simulink model "Powertrain"  (R2022a)
settings: Solver=FixedStepAuto  StartTime=0.0  StopTime=inf  FixedStep=1  RelTol=1e-3
model workspace (MAT data in the model file):
  Velocity_kmph = Simulink.Parameter
  Velocity_kmph.DataType = 'auto'
  Velocity_kmph.Complexity = 'real'
  Velocity_kmph.Dimensions = [0 0]
values from neighbouring files (symbols this model uses):
  Batt_Capacity = 66.2    [Imports.m]
  Batt_Energy = 24000    [Imports.m]
  Cd = 0.28    [Imports.m]
  Cell_SOC = Cell(:,3)    [Imports.m]
  Cell_Volt = Cell(:,2)    [Imports.m]
  Crf = 0.015    [Imports.m]
  Fa = 3.8056    [Imports.m]
  GR = 7.9377    [Imports.m]
  GVM = Mv+Md    (= 1710.665)    [Imports.m]
  GVW = GVM*g    (= 16781.62365)    [Imports.m]
  HSOC = 80    [Imports.m]
  Ir = 0.0023    [Imports.m]
  K_EMF = 0.238    [Imports.m]
  K_T = 0.195    [Imports.m]
  LSOC = 20    [Imports.m]
  M_C_Regen_Eff = M_C_Regen(:,2:16)    [Imports.m]
  M_C_Regen_Speed = M_C_Regen(:,1)    [Imports.m]
  M_C_Regen_Torque = M_C_Regen(:,17)    [Imports.m]
  M_Controller_Eff = M_Controller(:,2:16)    [Imports.m]
  M_Controller_Speed = M_Controller(:,1)    [Imports.m]
  M_Controller_Torque = M_Controller(:,17)    [Imports.m]
  Max_Battery_Regen_Current = Max_Regen_Current*Np    (= 66.2)    [Imports.m]
  Motor_Eff = Motor(:,2:16)    [Imports.m]
  Motor_Regen_Eff = Motor_Regen(:,2:16)    [Imports.m]
  Motor_Regen_Speed = Motor_Regen(:,1)    [Imports.m]
  Motor_Regen_Torque = Motor_Regen(:,17)    [Imports.m]
  Motor_Speed = Motor(:,1)    [Imports.m]
  Motor_Torque = Motor(:,17)    [Imports.m]
  Ns = 96    [Imports.m]
  R_Arm = 0.00567    [Imports.m]
  rho = 1.225    [Imports.m]
  Rw = 0.2032    [Imports.m]
  Teff = 0.89    [Imports.m]
settings Model: Creator=goodbox  LastModifiedBy=sujee
settings SolverCC: AlgebraicLoopSolver=TrustRegion
settings DebuggingCC: UnconnectedInputMsg=warning  UnconnectedOutputMsg=warning  UnconnectedLineMsg=warning  SFMachineParentedDataDiag=warning

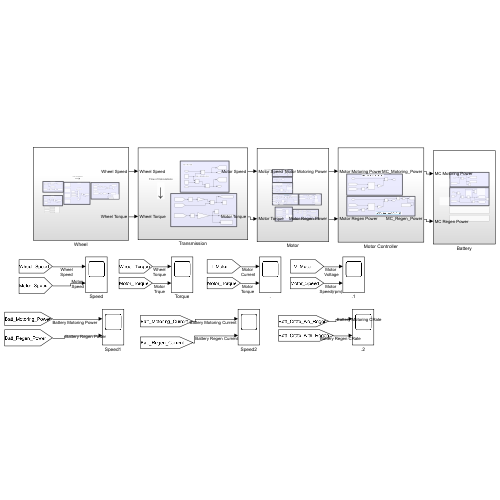
[thumbnail: Simulink's stored preview of the top-level diagram]
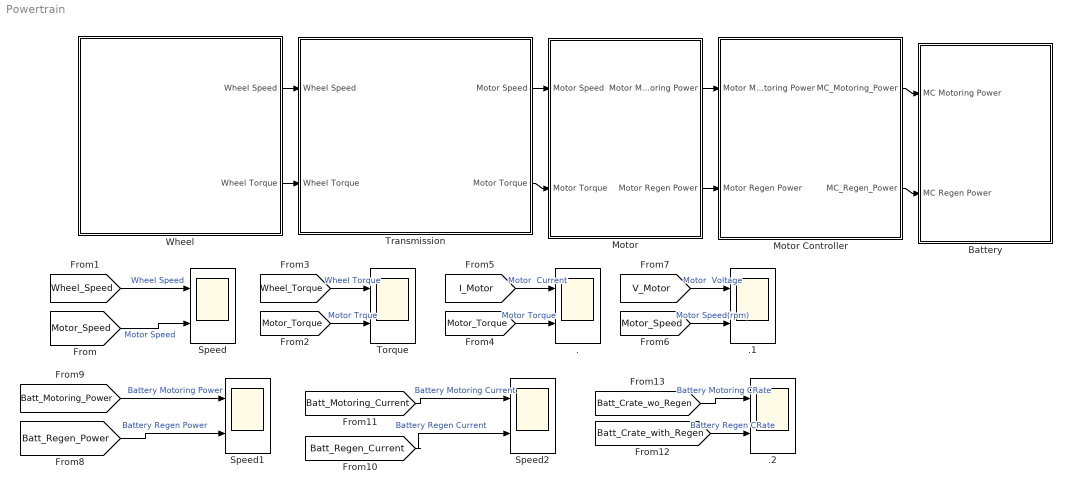
== system Powertrain ==
  . : Scope  NumInputPorts=2
  .1 : Scope  NumInputPorts=2
  .2 : Scope  NumInputPorts=2
  Battery : Subsystem
  Motor : Subsystem
  Motor Controller : Subsystem
  Speed : Scope  NumInputPorts=2
  Speed1 : Scope  NumInputPorts=2
  Speed2 : Scope  NumInputPorts=2
  Torque : Scope  NumInputPorts=2
  Transmission : Subsystem
  Wheel : Subsystem
  wires:
  Wheel/1(Wheel Speed) -> Transmission/1(Wheel Speed)
  Wheel/2(Wheel Torque) -> Transmission/2(Wheel Torque)
  [Wheel_Speed] -> Speed/1  "Wheel Speed"
  [Motor_Speed] -> Speed/2  "Motor Speed"
  [Motor_Torque] -> Torque/2  "Motor Trque"
  [Wheel_Torque] -> Torque/1  "Wheel Torque"
  Transmission/1(Motor Speed) -> Motor/1(Motor Speed)
  Transmission/2(Motor Torque) -> Motor/2(Motor Torque)
  [I_Motor] -> ./1  "Motor  Current"
  [Motor_Torque] -> ./2  "Motor Torque"
  [Motor_Speed] -> .1/2  "Motor Speed(rpm)"
  [V_Motor] -> .1/1  "Motor  Voltage"
  Motor/1(Motor Motoring Power) -> Motor Controller/1(Motor Motoring Power)
  Motor/2(Motor Regen Power) -> Motor Controller/2(Motor Regen Power)
  Motor Controller/2(MC_Regen_Power) -> Battery/2(MC Regen Power)
  Motor Controller/1(MC_Motoring_Power) -> Battery/1(MC Motoring Power)
  [Batt_Regen_Power] -> Speed1/2  "Battery Regen Power"
  [Batt_Motoring_Power] -> Speed1/1  "Battery Motoring Power"
  [Batt_Motoring_Current] -> Speed2/1  "Battery Motoring Current"
  [Batt_Regen_Current] -> Speed2/2  "Battery Regen Current"
  [Batt_Crate_wo_Regen] -> .2/1  "Battery Motoring CRate"
  [Batt_Crate_with_Regen] -> .2/2  "Battery Regen CRate"

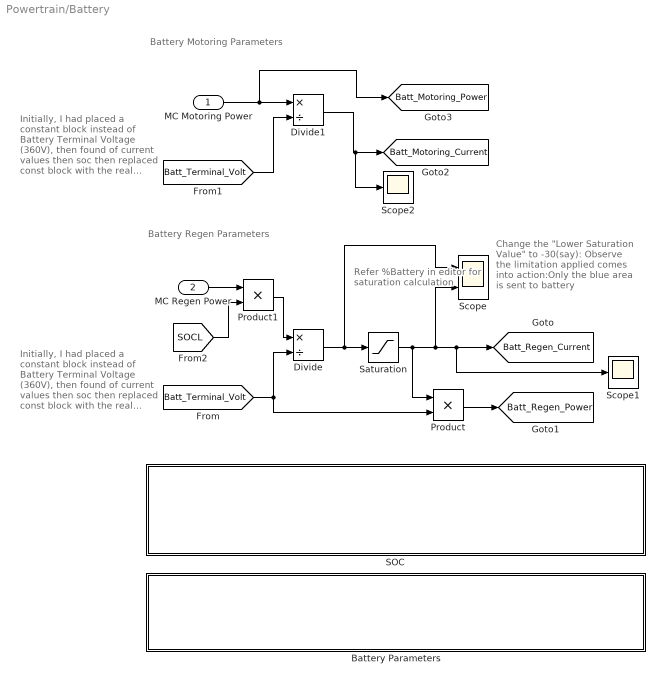
== system Powertrain/Battery ==
  note: Initially, I had placed a constant block instead of Battery Terminal Voltage (360V), then found of current values then soc then replaced const block with the real battery terminal voltage...
  note: Battery Motoring Parameters
  note: Battery Regen Parameters
  note: Refer %Battery in editor for saturation calculation
  note: Change the "Lower Saturation Value" to -30(say): Observe the limitation applied comes into action:Only the blue area is sent to battery
  note: Initially, I had placed a constant block instead of Battery Terminal Voltage (360V), then found of current values then soc then replaced const block with the real battery terminal voltage...
  MC Motoring Power : Inport
  MC Regen Power : Inport  Port=2
  Battery Parameters : Subsystem
  Divide : Product  Inputs=*/
  Divide1 : Product  Inputs=*/
  Product : Product
  Product1 : Product
  SOC : Subsystem
  Saturation : Saturate  UpperLimit=0  LowerLimit=-(Max_Battery_Regen_Current)
  Scope : Scope  NumInputPorts=2
  Scope1 : Scope
  Scope2 : Scope
  tag scope: Batt_Motoring_Current=global, Batt_Motoring_Power=global, Batt_Regen_Current=global, Batt_Regen_Power=global
  wires:
  [Batt_Terminal_Volt] -> Product/2, Divide/2
  Divide/1 -> Scope/1, Saturation/1
  Saturation/1 -> Scope/2, Scope1/1, [Batt_Regen_Current], Product/1
  Product/1 -> [Batt_Regen_Power]
  MC Motoring Power/1 -> [Batt_Motoring_Power], Divide1/1
  [Batt_Terminal_Volt] -> Divide1/2
  Divide1/1 -> Scope2/1, [Batt_Motoring_Current]
  Product1/1 -> Divide/1
  MC Regen Power/1 -> Product1/1
  [SOCL] -> Product1/2

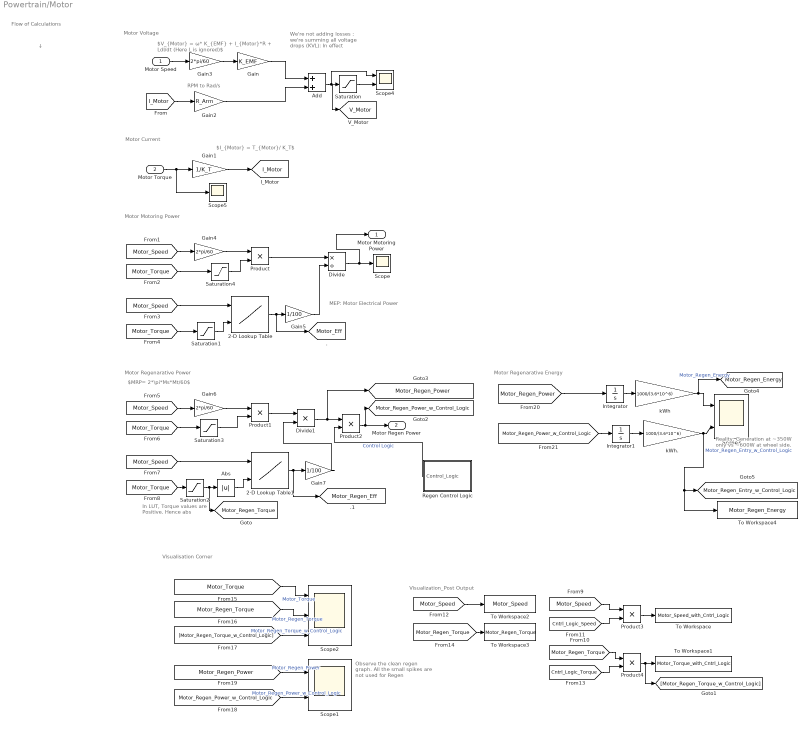
== system Powertrain/Motor ==
  note: Visualization_Post Output
  note: Motor Regenarative Energy
  note: Visualisation Corner
  note: Observe the clean regen graph. All the small spikes are not used for Regen
  note: MEP: Motor Electrical Power
  note: In LUT, Torque values are Positive. Hence abs
  note: $MRP= 2*\pi*Ms*Mt/60$
  note: Motor Motoring Power
  note: Motor Current
  note: Motor Voltage
  note: We're not adding losses : we're summing all voltage drops (KVL): In effect
  note: RPM to Rad/s
  note: $I_{Motor} = T_{Motor}/ K_T$
  note: $V_{Motor} = ω* K_{EMF} + I_{Motor}*R + LdI/dt (Here L is ignored)$
  note: Motor Regenarative Power
  note: ↓
  note: Flow of Calculations
  note: Reality: Generation at ~350W only vs ~600W at wheel side.
  Motor Speed : Inport
  Motor Torque : Inport  Port=2
  2-D Lookup Table : Lookup_n-D  BreakpointsForDimension1=Motor_Speed  BreakpointsForDimension2=Motor_Torque  Table=Motor_Eff  InternalRulePriority=Speed  RndMeth=Simplest
      settings: InputPortMap=u0,u1
  2-D Lookup Table1 : Lookup_n-D  BreakpointsForDimension1=Motor_Regen_Speed  BreakpointsForDimension2=Motor_Regen_Torque  Table=Motor_Regen_Eff  InternalRulePriority=Speed  RndMeth=Simplest
      settings: InputPortMap=u0,u1
  Abs : Abs  SaturateOnIntegerOverflow=off
  Add : Sum
  Divide : Product  Inputs=*/
  Divide1 : Product  Inputs=**
  Gain : Gain  Gain=K_EMF
  Gain1 : Gain  Gain=1/K_T
  Gain2 : Gain  Gain=R_Arm
  Gain3 : Gain  Gain=2*pi/60
  Gain4 : Gain  Gain=2*pi/60
  Gain5 : Gain  Gain=1/100
  Gain6 : Gain  Gain=2*pi/60
  Gain7 : Gain  Gain=1/100
  Integrator : Integrator
  Integrator1 : Integrator
  Product{,1..4} (5 alike) : Product
  Regen Control Logic : Subsystem
      settings: PortSchema="{\"entries\":[{\"content\":{\"sides\":[{\"content\":{\"connectorIds\":[\"Out1\"]},\"type\":\"ConnectorPlacement.EquallySpacedRectSide\",\"uuid\":\"9e0a81c3-7851-4a2a-9294-227ed6cb1b10\"},{\"content\":{\"connectorIds\":[],\"side\":\"RIGHT\"},\"type\":\"ConnectorPlacement.EquallySpacedRectSide\",\"uuid\":\"e9ef44a6-e013-44a9-929d-6b26e6cf2f5f\"},{\"content\":{\"connectorIds\":[],\"side\":\"TOP\"},\"type\":\"ConnectorPlacement.EquallySpacedRectSide\",\"uuid\":\"caa0c9f2-8ad3-43be-baf4-e18c04196c42\"}]},\"type\":\"ConnectorPlacement.EquallySpacedConnector\",\"uuid\":\"14208f40-628f-4a93-bd22-09b3f37d5a54\"}],\"packageUris\":[\"http://schema.mathworks.com/mf0/Connector/R2020b\"],\"version\":\"1.0\"}"
  Saturation : Saturate  UpperLimit=inf  LowerLimit=0
  Saturation1 : Saturate  UpperLimit=inf  LowerLimit=0
  Saturation2 : Saturate  UpperLimit=0  LowerLimit=-inf
  Saturation3 : Saturate  UpperLimit=0  LowerLimit=-inf
  Saturation4 : Saturate  UpperLimit=inf  LowerLimit=0
  Scope : Scope
  Scope1 : Scope  NumInputPorts=2
  Scope2 : Scope  NumInputPorts=3
  Scope3 : Scope  NumInputPorts=2
  Scope4 : Scope  NumInputPorts=2
  Scope5 : Scope
  To Workspace : ToWorkspace  VariableName=Motor_Speed_with_Cntrl_Logic  SaveFormat=Timeseries  SampleTime=-1
  To Workspace1 : ToWorkspace  VariableName=Motor_Torque_with_Cntrl_Logic  SaveFormat=Timeseries  SampleTime=-1
  To Workspace2 : ToWorkspace  VariableName=Motor_Speed  SaveFormat=Timeseries  SampleTime=-1
  To Workspace3 : ToWorkspace  VariableName=Motor_Regen_Torque  SaveFormat=Timeseries  SampleTime=-1
  To Workspace4 : ToWorkspace  VariableName=Motor_Regen_Energy  SaveFormat=Timeseries  SampleTime=-1
  kWh : Gain  Gain=1000/(3.6*10^6)
  kWh. : Gain  Gain=1000/(3.6*10^6)
  Motor Motoring Power : Outport
  Motor Regen Power : Outport  Port=2
  tag scope: I_Motor=global, Motor_Eff=global, Motor_Regen_Eff=global, Motor_Regen_Energy=global, Motor_Regen_Entry_w_Control_Logic=global, Motor_Regen_Power=global, Motor_Regen_Power_w_Control_Logic=global, Motor_Regen_Torque=global, V_Motor=global
  wires:
  Gain/1 -> Add/1
  Motor Torque/1 -> Scope5/1, Gain1/1
  Gain1/1 -> [I_Motor]
  [I_Motor] -> Gain2/1
  Gain2/1 -> Add/2
  Motor Speed/1 -> Gain3/1
  Gain3/1 -> Gain/1
  Add/1 -> Scope4/1, Saturation/1, [V_Motor]
  [Motor_Speed] -> Gain4/1
  Gain4/1 -> Product/1
  [Motor_Speed] -> 2-D Lookup Table/1
  2-D Lookup Table/1 -> [Motor_Eff], Gain5/1
  Product/1 -> Divide/1
  Gain5/1 -> Divide/2
  [Motor_Torque] -> Saturation1/1
  Saturation1/1 -> 2-D Lookup Table/2
  Divide/1 -> Scope/1, Motor Motoring Power/1
  [Motor_Speed] -> 2-D Lookup Table1/1
  Product1/1 -> Divide1/1
  2-D Lookup Table1/1 -> [Motor_Regen_Eff], Gain7/1
  [Motor_Torque] -> Saturation2/1
  Gain6/1 -> Product1/1
  Gain7/1 -> Divide1/2
  [Motor_Speed] -> Gain6/1
  Saturation2/1 -> [Motor_Regen_Torque], Abs/1
  Abs/1 -> 2-D Lookup Table1/2
  [Motor_Torque] -> Saturation3/1
  Saturation3/1 -> Product1/2
  Product2/1 -> [Motor_Regen_Power_w_Control_Logic], Motor Regen Power/1
  Regen Control Logic/1(Control_Logic) -> Product2/2  "Control Logic"
  Divide1/1 -> [Motor_Regen_Power], Product2/1
  [Motor_Regen_Torque] -> Product4/1
  [Cntrl_Logic_Torque] -> Product4/2
  [Cntrl_Logic_Speed] -> Product3/2
  [Motor_Speed] -> Product3/1
  Product3/1 -> To Workspace/1
  Product4/1 -> [Motor_Regen_Torque_w_Control_Logic], To Workspace1/1
  [Motor_Speed] -> To Workspace2/1
  [Motor_Regen_Torque] -> To Workspace3/1
  [Motor_Torque] -> Scope2/1  "Motor_Torque"
  [Motor_Regen_Torque] -> Scope2/2  "Motor_Regen_Torque"
  [Motor_Regen_Torque_w_Control_Logic] -> Scope2/3  "Motor_Regen_Torque_w_Control_Logic"
  [Motor_Regen_Power_w_Control_Logic] -> Scope1/2  "Motor_Regen_Power_w_Control_Logic"
  [Motor_Regen_Power] -> Scope1/1  "Motor_Regen_Power"
  kWh/1 -> [Motor_Regen_Energy], Scope3/1  "Motor_Regen_Energy"
  Integrator/1 -> kWh/1
  [Motor_Regen_Power] -> Integrator/1
  [Motor_Regen_Power_w_Control_Logic] -> Integrator1/1
  Integrator1/1 -> kWh./1
  kWh./1 -> To Workspace4/1, [Motor_Regen_Entry_w_Control_Logic], Scope3/2  "Motor_Regen_Entry_w_Control_Logic"
  Saturation/1 -> Scope4/2
  [Motor_Torque] -> Saturation4/1
  Saturation4/1 -> Product/2

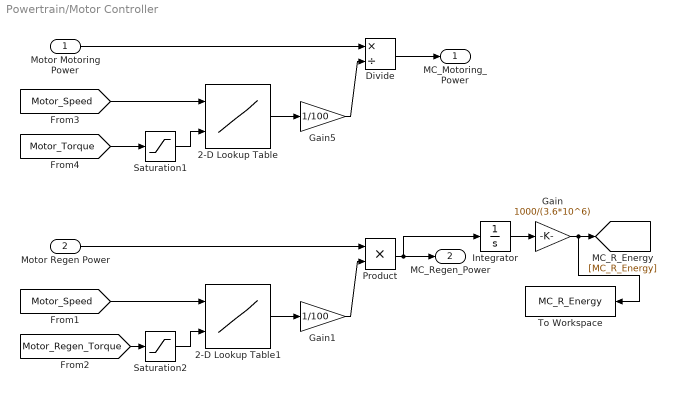
== system Powertrain/Motor Controller ==
  Motor Motoring Power : Inport
  Motor Regen Power : Inport  Port=2
  2-D Lookup Table : Lookup_n-D  BreakpointsForDimension1=M_Controller_Speed  BreakpointsForDimension2=M_Controller_Torque  Table=M_Controller_Eff  InternalRulePriority=Speed  RndMeth=Simplest
      settings: InputPortMap=u0,u1
  2-D Lookup Table1 : Lookup_n-D  BreakpointsForDimension1=M_C_Regen_Speed  BreakpointsForDimension2=M_C_Regen_Torque  Table=M_C_Regen_Eff  InternalRulePriority=Speed  RndMeth=Simplest
      settings: InputPortMap=u0,u1
  Divide : Product  Inputs=*/
  Gain : Gain  Gain=1000/(3.6*10^6)
  Gain1 : Gain  Gain=1/100
  Gain5 : Gain  Gain=1/100
  Integrator : Integrator
  Product : Product
  Saturation1 : Saturate  UpperLimit=inf  LowerLimit=0
  Saturation2 : Saturate  UpperLimit=inf  LowerLimit=0
  To Workspace : ToWorkspace  VariableName=MC_R_Energy  SaveFormat=Timeseries  SampleTime=-1
  MC_Motoring_Power : Outport
  MC_Regen_Power : Outport  Port=2
  wires:
  2-D Lookup Table/1 -> Gain5/1
  [Motor_Speed] -> 2-D Lookup Table/1
  Saturation1/1 -> 2-D Lookup Table/2
  [Motor_Torque] -> Saturation1/1
  [Motor_Regen_Torque] -> Saturation2/1
  Saturation2/1 -> 2-D Lookup Table1/2
  [Motor_Speed] -> 2-D Lookup Table1/1
  2-D Lookup Table1/1 -> Gain1/1
  Motor Motoring Power/1 -> Divide/1
  Motor Regen Power/1 -> Product/1
  Gain1/1 -> Product/2
  Gain5/1 -> Divide/2
  Divide/1 -> MC_Motoring_Power/1
  Product/1 -> MC_Regen_Power/1, Integrator/1
  Integrator/1 -> Gain/1
  Gain/1 -> [MC_R_Energy], To Workspace/1

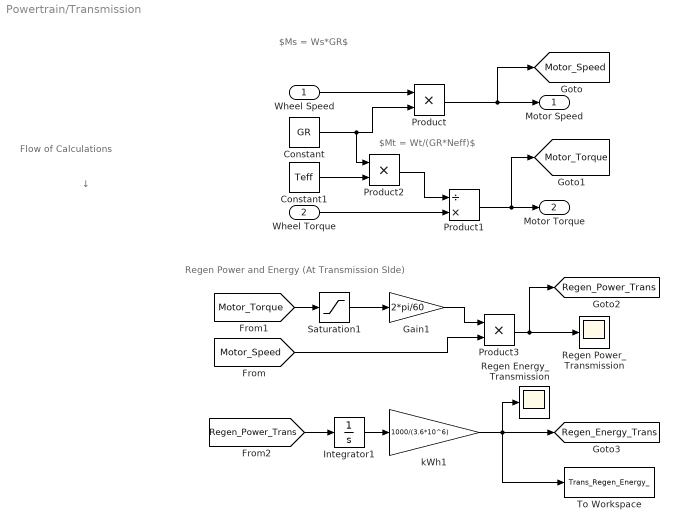
== system Powertrain/Transmission ==
  note: ↓
  note: Regen Power and Energy (At Transmission SIde)
  note: $Mt = Wt/(GR*Neff)$
  note: $Ms = Ws*GR$
  note: Flow of Calculations
  Wheel Speed : Inport
  Wheel Torque : Inport  Port=2
  Constant : Constant  Value=GR
  Constant1 : Constant  Value=Teff
  Gain1 : Gain  Gain=2*pi/60
  Integrator1 : Integrator
  Product : Product
  Product1 : Product  Inputs=/*
  Product2 : Product
  Product3 : Product
  Regen Energy_Transmission : Scope
  Regen Power_Transmission : Scope
  Saturation1 : Saturate  UpperLimit=0  LowerLimit=-inf
  To Workspace : ToWorkspace  VariableName=Trans_Regen_Energy_  SaveFormat=Timeseries  SampleTime=-1
  kWh1 : Gain  Gain=1000/(3.6*10^6)
  Motor Speed : Outport
  Motor Torque : Outport  Port=2
  tag scope: Motor_Speed=global, Motor_Torque=global, Regen_Energy_Trans=global, Regen_Power_Trans=global
  wires:
  Wheel Speed/1 -> Product/1
  Constant/1 -> Product2/1, Product/2
  Product/1 -> [Motor_Speed], Motor Speed/1
  Constant1/1 -> Product2/2
  Wheel Torque/1 -> Product1/2
  Product2/1 -> Product1/1
  Product1/1 -> [Motor_Torque], Motor Torque/1
  Integrator1/1 -> kWh1/1
  kWh1/1 -> To Workspace/1, [Regen_Energy_Trans], Regen Energy_Transmission/1
  [Regen_Power_Trans] -> Integrator1/1
  Gain1/1 -> Product3/1
  [Motor_Torque] -> Saturation1/1
  [Motor_Speed] -> Product3/2
  Saturation1/1 -> Gain1/1
  Product3/1 -> [Regen_Power_Trans], Regen Power_Transmission/1

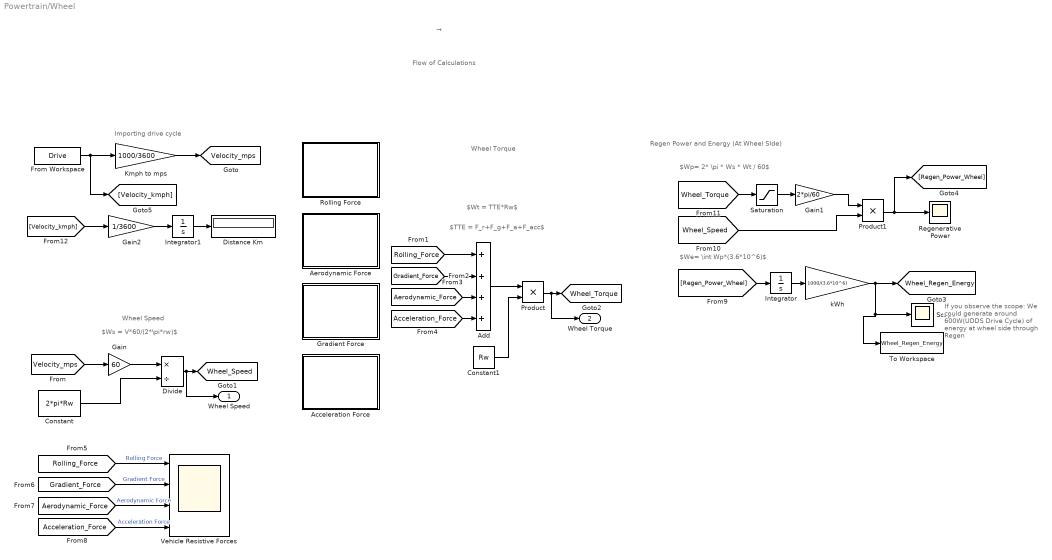
== system Powertrain/Wheel ==
  note: Flow of Calculations
  note: →
  note: $TTE = F_r+F_g+F_a+F_acc$
  note: $Wt = TTE*Rw$
  note: Wheel Torque
  note: $Ws = V*60/(2*\pi*rw)$
  note: Wheel Speed
  note: Importing drive cycle
  note: Regen Power and Energy (At Wheel SIde)
  note: $We= \int Wp*(3.6*10^6)$
  note: $Wp= 2* \pi * Ws * Wt / 60$
  note: If you observe the scope: We could generate around 600W(UDDS Drive Cycle) of energy at wheel side through Regen
  Acceleration Force : Subsystem
  Add : Sum  Inputs=4
  Aerodynamic Force : Subsystem
  Constant : Constant  Value=2*pi*Rw
  Constant1 : Constant  Value=Rw
  Distance Km : Display
  Divide : Product  Inputs=*/
  From Workspace : FromWorkspace  VariableName=Drive
  Gain : Gain  Gain=60
  Gain1 : Gain  Gain=2*pi/60
  Gain2 : Gain  Gain=1/3600
  Gradient Force : Subsystem
  Integrator : Integrator
  Integrator1 : Integrator
  Kmph to mps : Gain  Gain=1000/3600
  Product : Product
  Product1 : Product
  Regenerative Power : Scope
  Rolling Force : Subsystem
  Saturation : Saturate  UpperLimit=0  LowerLimit=-inf
  Scope : Scope
  To Workspace : ToWorkspace  VariableName=Wheel_Regen_Energy  SaveFormat=Timeseries  SampleTime=-1
  Vehicle Resistive Forces : Scope  NumInputPorts=4
  kWh : Gain  Gain=1000/(3.6*10^6)
  Wheel Speed : Outport
  Wheel Torque : Outport  Port=2
  tag scope: Velocity_mps=global, Wheel_Regen_Energy=global, Wheel_Speed=global, Wheel_Torque=global
  wires:
  From Workspace/1 -> [Velocity_kmph], Kmph to mps/1
  Kmph to mps/1 -> [Velocity_mps]
  [Velocity_mps] -> Gain/1
  Gain/1 -> Divide/1
  Constant/1 -> Divide/2
  Divide/1 -> Wheel Speed/1, [Wheel_Speed]
  [Rolling_Force] -> Add/1
  [Gradient_Force] -> Add/2
  [Aerodynamic_Force] -> Add/3
  [Acceleration_Force] -> Add/4
  Add/1 -> Product/1
  Constant1/1 -> Product/2
  Product/1 -> Wheel Torque/1, [Wheel_Torque]
  [Rolling_Force] -> Vehicle Resistive Forces/1  "Rolling Force"
  [Gradient_Force] -> Vehicle Resistive Forces/2  "Gradient Force"
  [Aerodynamic_Force] -> Vehicle Resistive Forces/3  "Aerodynamic Force"
  [Acceleration_Force] -> Vehicle Resistive Forces/4  "Acceleration Force"
  Saturation/1 -> Gain1/1
  Gain1/1 -> Product1/1
  Product1/1 -> [Regen_Power_Wheel], Regenerative Power/1
  [Wheel_Torque] -> Saturation/1
  [Wheel_Speed] -> Product1/2
  kWh/1 -> [Wheel_Regen_Energy], To Workspace/1, Scope/1
  Integrator/1 -> kWh/1
  [Regen_Power_Wheel] -> Integrator/1
  [Velocity_kmph] -> Gain2/1
  Gain2/1 -> Integrator1/1
  Integrator1/1 -> Distance Km/1

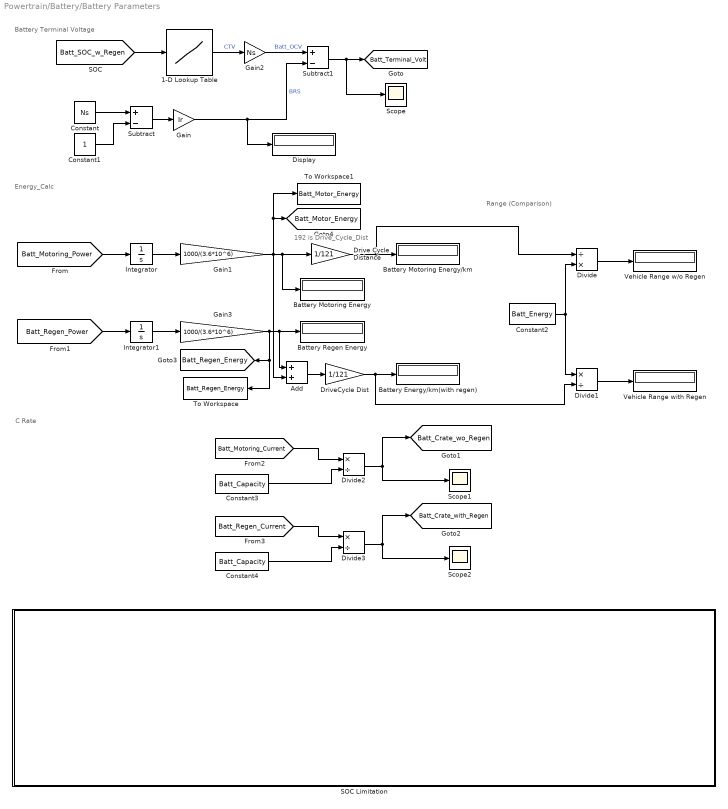
== system Powertrain/Battery/Battery Parameters ==
  note: 192 is Drive_Cycle_Dist
  note: C Rate
  note: Range (Comparison)
  note: Energy_Calc
  note: Battery Terminal Voltage
  1-D Lookup Table : Lookup_n-D  NumberOfTableDimensions=1  BreakpointsForDimension1=Cell_SOC  Table=Cell_Volt  InternalRulePriority=Speed  RndMeth=Simplest
  Add : Sum
  Battery Energy/km(with regen) : Display
  Battery Motoring Energy : Display
  Battery Motoring Energy/km : Display
  Battery Regen Energy : Display
  Constant : Constant  Value=Ns
  Constant1 : Constant
  Constant2 : Constant  Value=Batt_Energy
  Constant3 : Constant  Value=Batt_Capacity
  Constant4 : Constant  Value=Batt_Capacity
  Display : Display
  Divide : Product  Inputs=/*
  Divide1 : Product  Inputs=*/
  Divide2 : Product  Inputs=*/
  Divide3 : Product  Inputs=*/
  Drive Cycle Distance : Gain  Gain=1/121
  DriveCycle Dist : Gain  Gain=1/121
  Gain : Gain  Gain=Ir
  Gain1 : Gain  Gain=1000/(3.6*10^6)
  Gain2 : Gain  Gain=Ns
  Gain3 : Gain  Gain=1000/(3.6*10^6)
  Integrator : Integrator
  Integrator1 : Integrator
  SOC Limitation : Subsystem
  Scope : Scope
  Scope1 : Scope
  Scope2 : Scope
  Subtract : Sum  Inputs=+-
  Subtract1 : Sum  Inputs=+-
  To Workspace : ToWorkspace  VariableName=Batt_Regen_Energy  SaveFormat=Timeseries  SampleTime=-1
  To Workspace1 : ToWorkspace  VariableName=Batt_Motor_Energy  SaveFormat=Timeseries  SampleTime=-1
  Vehicle Range w/o Regen : Display
  Vehicle Range with Regen : Display
  tag scope: Batt_Crate_with_Regen=global, Batt_Crate_wo_Regen=global, Batt_Motor_Energy=global, Batt_Regen_Energy=global, Batt_Terminal_Volt=global
  wires:
  1-D Lookup Table/1 -> Gain2/1  "CTV"
  Subtract1/1 -> Scope/1, [Batt_Terminal_Volt]
  Constant1/1 -> Subtract/2
  [Batt_SOC_w_Regen] -> 1-D Lookup Table/1
  Constant/1 -> Subtract/1
  Gain/1 -> Display/1, Subtract1/2  "BRS"
  Gain2/1 -> Subtract1/1  "Batt_OCV"
  Subtract/1 -> Gain/1
  [Batt_Motoring_Power] -> Integrator/1
  [Batt_Regen_Power] -> Integrator1/1
  Integrator/1 -> Gain1/1
  Integrator1/1 -> Gain3/1
  Gain1/1 -> To Workspace1/1, [Batt_Motor_Energy], Add/2, Drive Cycle Distance/1, Battery Motoring Energy/1
  Gain3/1 -> To Workspace/1, [Batt_Regen_Energy], Battery Regen Energy/1, Add/1
  Drive Cycle Distance/1 -> Divide/1, Battery Motoring Energy/km/1
  Add/1 -> DriveCycle Dist/1
  DriveCycle Dist/1 -> Divide1/2, Battery Energy/km(with regen)/1
  Divide/1 -> Vehicle Range w/o Regen/1
  Divide1/1 -> Vehicle Range with Regen/1
  Constant2/1 -> Divide1/1, Divide/2
  [Batt_Motoring_Current] -> Divide2/1
  Constant3/1 -> Divide2/2
  Divide2/1 -> [Batt_Crate_wo_Regen], Scope1/1
  Divide3/1 -> Scope2/1, [Batt_Crate_with_Regen]
  Constant4/1 -> Divide3/2
  [Batt_Regen_Current] -> Divide3/1

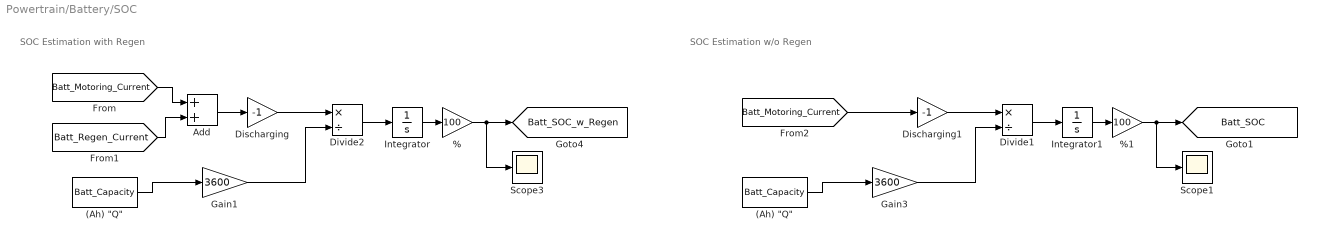
== system Powertrain/Battery/SOC ==
  note: SOC Estimation with Regen
  note: SOC Estimation w/o Regen
  " (Ah) \"Q\"" : Constant  Value=Batt_Capacity
  % : Gain  Gain=100
  %1 : Gain  Gain=100
  "(Ah) \"Q\"" : Constant  Value=Batt_Capacity
  Add : Sum
  Discharging : Gain  Gain=-1
  Discharging1 : Gain  Gain=-1
  Divide1 : Product  Inputs=*/
  Divide2 : Product  Inputs=*/
  Gain1 : Gain  Gain=3600
  Gain3 : Gain  Gain=3600
  Integrator : Integrator  InitialCondition=1
  Integrator1 : Integrator  InitialCondition=1
  Scope1 : Scope
  Scope3 : Scope
  tag scope: Batt_SOC=global, Batt_SOC_w_Regen=global
  wires:
  [Batt_Motoring_Current] -> Add/1
  %/1 -> Scope3/1, [Batt_SOC_w_Regen]
  Gain1/1 -> Divide2/2
  [Batt_Regen_Current] -> Add/2
  Integrator/1 -> %/1
  Add/1 -> Discharging/1
  "(Ah) \"Q\""/1 -> Gain1/1
  Divide2/1 -> Integrator/1
  Discharging/1 -> Divide2/1
  Discharging1/1 -> Divide1/1
  [Batt_Motoring_Current] -> Discharging1/1
  " (Ah) \"Q\""/1 -> Gain3/1
  %1/1 -> Scope1/1, [Batt_SOC]
  Divide1/1 -> Integrator1/1
  Gain3/1 -> Divide1/2
  Integrator1/1 -> %1/1

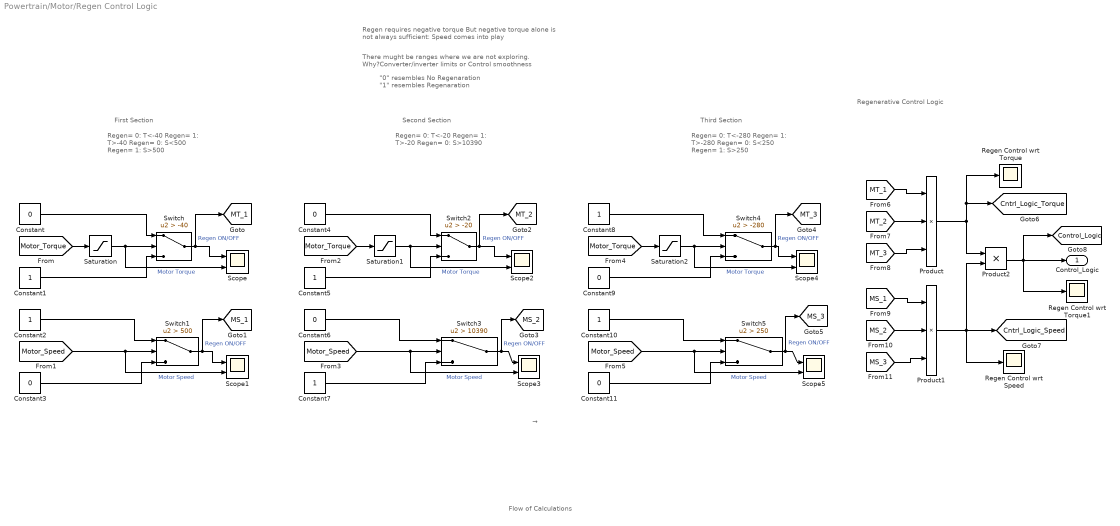
== system Powertrain/Motor/Regen Control Logic ==
  note: Regenerative Control Logic
  note: Regen requires negative torque
      | But negative torque alone is not always sufficient: Speed comes into play
  note: Regen= 0: T<-40
      | Regen= 1: T>-40
      |
      | Regen= 0: S<500
      | Regen= 1: S>500
  note: First Section
  note: There mught be ranges where we are not exploring.
      | Why?Converter/inverter limits or Control smoothness
  note: "0" resembles No Regenaration
      | "1" resembles  Regenaration
  note: Second Section
  note: Regen= 0: T<-20
      | Regen= 1: T>-20
      |
      | Regen= 0: S>10390
  note: Regen= 0: T<-280
      | Regen= 1: T>-280
      |
      | Regen= 0: S<250
      | Regen= 1: S>250
  note: Third Section
  note: →
  note: Flow of Calculations
  Constant{,3..4,6,9,11} (6 alike) : Constant  Value=0
  Constant{1..2,5,7..8,10} (6 alike) : Constant
  Product : Product  Inputs=3
  Product1 : Product  Inputs=3
  Product2 : Product
  Regen Control wrt Speed : Scope
  Regen Control wrt Torque : Scope
  Regen Control wrt Torque1 : Scope
  Saturation : Saturate  UpperLimit=0  LowerLimit=-inf
  Saturation1 : Saturate  UpperLimit=0  LowerLimit=-inf
  Saturation2 : Saturate  UpperLimit=0  LowerLimit=-inf
  Scope{,1..5} (6 alike) : Scope  NumInputPorts=2
  Switch : Switch  Criteria=u2 > Threshold  Threshold=-40  SaturateOnIntegerOverflow=off  InputSameDT=off
  Switch1 : Switch  Criteria=u2 > Threshold  Threshold=500  SaturateOnIntegerOverflow=off  InputSameDT=off
  Switch2 : Switch  Criteria=u2 > Threshold  Threshold=-20  SaturateOnIntegerOverflow=off  InputSameDT=off
  Switch3 : Switch  Criteria=u2 > Threshold  Threshold=10390  SaturateOnIntegerOverflow=off  InputSameDT=off
  Switch4 : Switch  Criteria=u2 > Threshold  Threshold=-280  SaturateOnIntegerOverflow=off  InputSameDT=off
  Switch5 : Switch  Criteria=u2 > Threshold  Threshold=250  SaturateOnIntegerOverflow=off  InputSameDT=off
  Control_Logic : Outport
  tag scope: Cntrl_Logic_Speed=global, Cntrl_Logic_Torque=global, Control_Logic=global, MS_1=global, MS_2=global, MS_3=global, MT_1=global, MT_2=global, MT_3=global
  wires:
  [Motor_Torque] -> Saturation/1
  Constant/1 -> Switch/1
  Constant1/1 -> Switch/3
  Switch/1 -> [MT_1], Scope/1  "Regen ON/OFF"
  Saturation/1 -> Scope/2, Switch/2  "Motor Torque"
  [Motor_Speed] -> Scope1/2, Switch1/2  "Motor Speed"
  Constant3/1 -> Switch1/3
  Switch1/1 -> [MS_1], Scope1/1  "Regen ON/OFF"
  Constant2/1 -> Switch1/1
  Saturation1/1 -> Scope2/2, Switch2/2  "Motor Torque"
  Switch3/1 -> [MS_2], Scope3/1  "Regen ON/OFF"
  Constant6/1 -> Switch3/1
  Constant7/1 -> Switch3/3
  [Motor_Speed] -> Scope3/2, Switch3/2  "Motor Speed"
  Constant5/1 -> Switch2/3
  Switch2/1 -> [MT_2], Scope2/1  "Regen ON/OFF"
  [Motor_Torque] -> Saturation1/1
  Constant4/1 -> Switch2/1
  [Motor_Speed] -> Scope5/2, Switch5/2  "Motor Speed"
  Constant11/1 -> Switch5/3
  Constant10/1 -> Switch5/1
  Saturation2/1 -> Scope4/2, Switch4/2  "Motor Torque"
  Switch5/1 -> [MS_3], Scope5/1  "Regen ON/OFF"
  Constant8/1 -> Switch4/1
  [Motor_Torque] -> Saturation2/1
  Switch4/1 -> [MT_3], Scope4/1  "Regen ON/OFF"
  Constant9/1 -> Switch4/3
  [MT_1] -> Product/1
  [MT_2] -> Product/2
  [MT_3] -> Product/3
  Product/1 -> Product2/1, Regen Control wrt Torque/1, [Cntrl_Logic_Torque]
  Product1/1 -> [Cntrl_Logic_Speed], Product2/2, Regen Control wrt Speed/1
  [MS_2] -> Product1/2
  [MS_1] -> Product1/1
  [MS_3] -> Product1/3
  Product2/1 -> Regen Control wrt Torque1/1, [Control_Logic], Control_Logic/1

== system Powertrain/Wheel/Acceleration Force ==
  note: $Facc = GVM*a$
  Constant : Constant  Value=GVM
  Derivative : Derivative
  Product : Product
  tag scope: Acceleration_Force=global
  wires:
  [Velocity_mps] -> Derivative/1
  Constant/1 -> Product/1
  Derivative/1 -> Product/2
  Product/1 -> [Acceleration_Force]

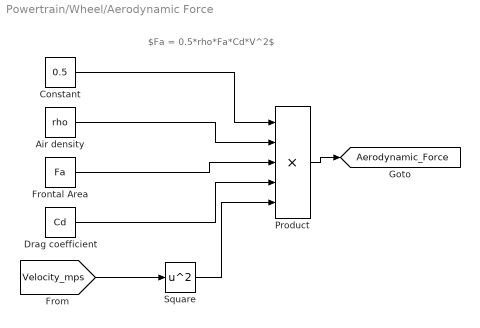
== system Powertrain/Wheel/Aerodynamic Force ==
  note: $Fa = 0.5*rho*Fa*Cd*V^2$
  Air density : Constant  Value=rho
  Constant : Constant  Value=0.5
  Drag coefficient : Constant  Value=Cd
  Frontal Area : Constant  Value=Fa
  Product : Product  Inputs=5
  Square : Math  Operator=square
  tag scope: Aerodynamic_Force=global
  wires:
  [Velocity_mps] -> Square/1
  Square/1 -> Product/5
  Drag coefficient/1 -> Product/4
  Frontal Area/1 -> Product/3
  Air density/1 -> Product/2
  Constant/1 -> Product/1
  Product/1 -> [Aerodynamic_Force]

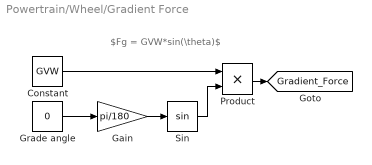
== system Powertrain/Wheel/Gradient Force ==
  note: $Fg = GVW*sin(\theta)$
  Constant : Constant  Value=GVW
  Gain : Gain  Gain=pi/180
  Grade angle : Constant  Value=0
  Product : Product
  Sin : Trigonometry
  tag scope: Gradient_Force=global
  wires:
  Grade angle/1 -> Gain/1
  Gain/1 -> Sin/1
  Constant/1 -> Product/1
  Sin/1 -> Product/2
  Product/1 -> [Gradient_Force]

== system Powertrain/Wheel/Rolling Force ==
  note: $Fr = GVW*Crf$
  Constant : Constant  Value=GVW
  Constant1 : Constant  Value=Crf
  Product : Product
  tag scope: Rolling_Force=global
  wires:
  Constant/1 -> Product/1
  Constant1/1 -> Product/2
  Product/1 -> [Rolling_Force]

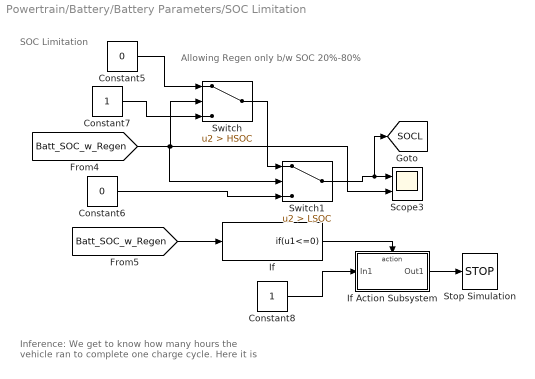
== system Powertrain/Battery/Battery Parameters/SOC Limitation ==
  note: Inference: We get to know how many hours the vehicle ran to complete one charge cycle. Here it is
  note: SOC Limitation
  note: Allowing Regen only b/w SOC 20%-80%
  Constant5 : Constant  Value=0
  Constant6 : Constant  Value=0
  Constant7 : Constant
  Constant8 : Constant
  If : If  IfExpression=u1<=0  ShowElse=off
  If Action Subsystem : Subsystem  TreatAsAtomicUnit=on
  Scope3 : Scope  NumInputPorts=2
  Stop Simulation : Stop
  Switch : Switch  Criteria=u2 > Threshold  Threshold=HSOC  SaturateOnIntegerOverflow=off  InputSameDT=off
  Switch1 : Switch  Criteria=u2 > Threshold  Threshold=LSOC  SaturateOnIntegerOverflow=off  InputSameDT=off
  tag scope: SOCL=global
  wires:
  [Batt_SOC_w_Regen] -> If/1
  If Action Subsystem/1(Out1) -> Stop Simulation/1
  Constant8/1 -> If Action Subsystem/1(In1)
  If/1 -> If Action Subsystem/Action
  Constant7/1 -> Switch/3
  Switch1/1 -> [SOCL], Scope3/1
  Switch/1 -> Switch1/1
  Constant5/1 -> Switch/1
  Constant6/1 -> Switch1/3
  [Batt_SOC_w_Regen] -> Scope3/2, Switch/2, Switch1/2

== system Powertrain/Battery/Battery Parameters/SOC Limitation/If Action Subsystem ==
  In1 : Inport
  Action Port : ActionPort  ActionPortLabel=if(u1<=0)
  Out1 : Outport
  wires:
  In1/1 -> Out1/1
